simulink model "reduce_emf_load_fixed_v13"  (R2024b)
settings: Solver=FixedStepAuto  StartTime=0.0  StopTime=25  FixedStep=Tsim  RelTol=1e-4  EnableMultiTasking=on
InitFcn:
  | clc;
  | clear;
  | %% Parameters of the motor
  | Tsim = 1e-6;
  | Tpwm=1e-4;
  | Ts = 1e-4;
  | R = 1.8665;
  | Rs=1.8665;
  | Ls=8.96e-3;
  | Ld = 8.96e-3;
  | Lq = 8.96e-3;
  | L1=(Ld +Lq )/2;
  | L2=(Lq -Ld )/2;
  | flux = 0.21;
  | F=0.00008;
  | J=0.003;
  | Np=4;
  | fpwm = 10e3;
  | Vdc=311;
  | wn=100;
  | %% Controller limiter                                                           % Maximum torque (Nm)
  | I_max = 7.5;                                                    % Maximum current (A)
  | V_max = Vdc/sqrt(3);
  | 
  | 
  | %% 转速环电流环带宽
  | wspd=20;
  | wcur=500;
  | 
  | %% LESO
  | w0=10000;
  | beta1=2*w0-R/Ld;
  | beta2=w0*w0;
  | %% IF启动
  | Iq_if=7;
  | we_if_acc=300;
  | we_if_max=180;
  | we_switch=150;
model workspace (MAT data in the model file):
  new = 0
undefined symbols (not defined in the file or in its folder): DiscIntNeverNeededParam
libraries: spsDCVoltageSourceLib x1, spsGroundLib x1, spsPermanentMagnetSynchronousMachineLib x1, spsUniversalBridgeLib x1, spspowerguiLib x1, simulink x1
(part 1 of 2)
settings Model: SimulationMode=accelerator  Creator=Lenovo  LastModifiedBy=azx
settings SolverCC: AlgebraicLoopSolver=TrustRegion
settings DataIOCC: ReturnWorkspaceOutputs=off
settings OptimizationCC: ReuseModelBlockBuffer=off
settings DebuggingCC: UnconnectedInputMsg=warning  UnconnectedOutputMsg=warning  UnconnectedLineMsg=warning
settings ModelReferenceCC: EnableRefExpFcnMdlSchedulingChecks=on
settings RTWCC: GPUComputeCapability=3.5

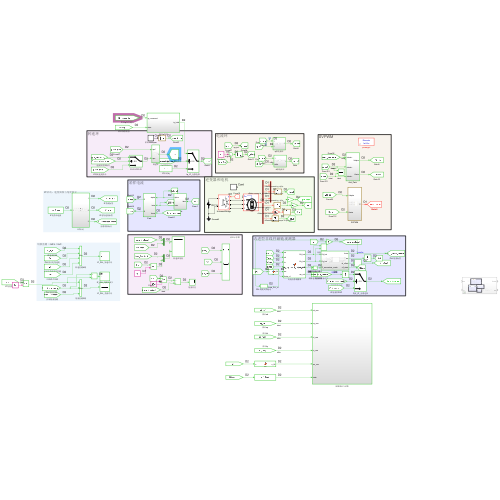
[thumbnail: Simulink's stored preview of the top-level diagram]
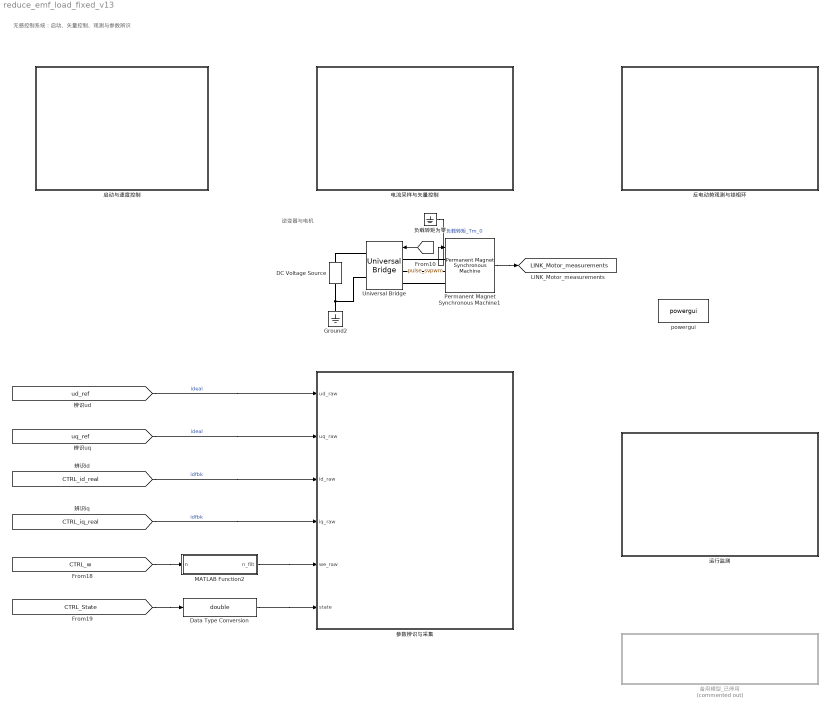
== system reduce_emf_load_fixed_v13 ==
  note: 无感控制系统：启动、矢量控制、观测与参数辨识
  note: 逆变器与电机
  DC Voltage Source : spsDCVoltageSourceLib/DC Voltage Source  Amplitude=Vdc  Measurements=None
  Data Type Conversion : DataTypeConversion  OutDataTypeStr=double  SaturateOnIntegerOverflow=off  RndMeth=Floor
  Ground2 : spsGroundLib/Ground  LConnTagsString=a
  MATLAB Function2 : MATLAB Function  TreatAsAtomicUnit=on
  Permanent Magnet Synchronous Machine1 : spsPermanentMagnetSynchronousMachineLib/Permanent Magnet Synchronous Machine  NbPhases=3  FluxDistribution=Sinusoidal  RotorType=Salient-pole  MechanicalLoad=Torque Tm  PresetModel=No  ShowDetailedParameters=on  MeasurementBus=off  Resistance=R  Inductance=8.5e-3  dqInductances=[Ld,Lq]  La=Ld  MachineConstant=Flux linkage established by magnets (V.s)  Flux=0.21  VoltageCst=152.3591  TorqueCst=1.26  Flat=120  Mechanical=[0.03 2e-2 Np 0]  PolePairs=4  InitialConditions=[0,0, 0,0]  InitialConditions5ph=[0 0 0 0 0 0]  RefAngle=Aligned with phase A axis (original Park)  IterativeDiscreteModel=Trapezoidal non iterative  TsBlock=-1  TsPowergui=0
  Universal Bridge : spsUniversalBridgeLib/Universal Bridge  Arms=3  SnubberResistance=1e5  SnubberCapacitance=inf  Device=IGBT / Diodes  Ron=1e-3  Lon=0  ForwardVoltages="[  0  0  ]"  ForwardVoltage=0  GTOparameters=[ 10e-6 , 20e-6 ]  IGBTparameters=[ 1e-6 , 2e-6 ]  Measurements=None  Measurements_2=None  converterType=Rectifier
  powergui : spspowerguiLib/powergui  Priority=1  SimulationMode=Discrete  SampleTime=Tsim  frequency=60  Iterations=50  frequencyindice=0  Pbase=100e6  ErrMax=1e-4  UnitsV=kV  UnitsW=MW  buscounter=0  FunctionMessages=off  echomessages=off  EnableUseOfTLC=off  CurrentSourceSwitches=off  DisableSnubberDevices=off  DisableRonSwitches=off  DisableVfSwitches=off  DisplayEquations=off  AutomaticDiscreteSolvers=off  SolverType=Tustin/Backward Euler (TBE)  Interpol=off  ExternalGateDelay=off  methode=off  Ts=100  x0status=blocks  SPID=on  SwTol=0  HookPort=off  NonlinearTolerance=1e-4  nMaxIteration=100  ContinueOnMaxIteration=off  RestoreLinks=warning  ResistiveCurrentMeasurement=off  Frange=[0:2:500]  Ylog=off  Xlog=on  ShowGrid=off  save=off  variable=ZData  structure=0  ZoomFFT=off  StartTime=0.0  cycles=1  DisplayStyle=1  fundamental=60  FreqAxis=off  MaxFrequency=1000  frequencyindicesteady=1  RmsSteady=1  display=off
  参数辨识与采集 : Subsystem
  启动与速度控制 : Subsystem  Description=仅整理原计算块与信号标签；虚拟子系统，不增加采样、延迟或执行条件。
  电流采样与矢量控制 : Subsystem  Description=仅整理原计算块与信号标签；虚拟子系统，不增加采样、延迟或执行条件。
  反电动势观测与锁相环 : Subsystem  Description=仅整理原计算块与信号标签；虚拟子系统，不增加采样、延迟或执行条件。
  运行监测 : Subsystem  Description=仅整理原计算块与信号标签；虚拟子系统，不增加采样、延迟或执行条件。
  负载转矩为零 : Ground
  备用模型_已停用 : Subsystem  Commented=on
  tag scope: LINK_Motor_measurements=global
  wires:
  [pulse_svpwm] -> Universal Bridge/1
  Permanent Magnet Synchronous Machine1/1 -> [LINK_Motor_measurements]
  [CTRL_w] -> MATLAB Function2/1(n)
  [CTRL_State] -> Data Type Conversion/1
  [ud_ref] -> 参数辨识与采集/1(ud_raw)  "ideal"
  [uq_ref] -> 参数辨识与采集/2(uq_raw)  "ideal"
  [CTRL_id_real] -> 参数辨识与采集/3(id_raw)  "idfbk"
  [CTRL_iq_real] -> 参数辨识与采集/4(iq_raw)  "idfbk"
  MATLAB Function2/1(n_filt) -> 参数辨识与采集/5(we_raw)
  Data Type Conversion/1 -> 参数辨识与采集/6(state)
  负载转矩为零/1 -> Permanent Magnet Synchronous Machine1/1  "负载转矩_Tm_0"
  connections:
  DC Voltage Source/RConn1 -- Universal Bridge/RConn1
  Permanent Magnet Synchronous Machine1/LConn1 -- Universal Bridge/LConn1
  Permanent Magnet Synchronous Machine1/LConn2 -- Universal Bridge/LConn2
  Permanent Magnet Synchronous Machine1/LConn3 -- Universal Bridge/LConn3
  Universal Bridge/RConn2 -- DC Voltage Source/LConn1 -- Ground2/LConn1

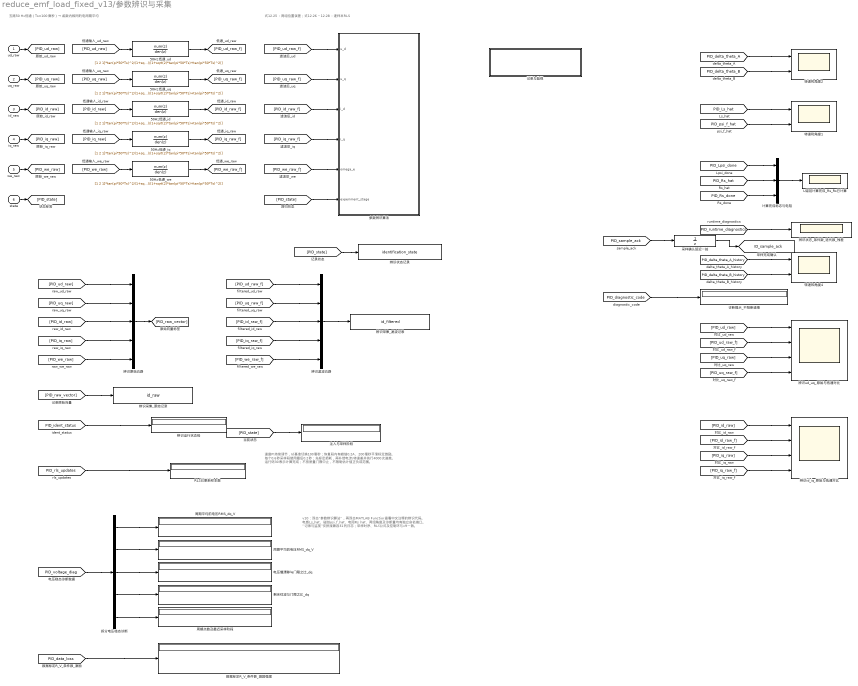
== system reduce_emf_load_fixed_v13/参数辨识与采集 ==
  note: 五路50 Hz低通（Ts=100微秒）→ 函数内相同的电周期平均
  note: 式12.25：两组位置误差；式12.26～12.28：逐样本RLS
  note: 速度PI持续调节，Id基准切换100毫秒；恢复段内有峰值0.2A、200毫秒平滑标定激励。
      | 每个0.6秒采样段使用最后0.2秒；先标定损耗，再补偿电流/转速差并执行4000次递推。
      | 运行码30表示计算完成；不按质量门限中止，不限制估计值正负或范围。
  note: v10：双击“参数辨识算法”，再双击MATLAB Function查看中文注释的辨识代码。
      | 电感Ls_hat、磁链psi_f_hat、电阻Rs_hat、两组角度及诊断量均有独立命名端口。
      | “记录与监视”仅拼接兼容31列日志；采样时序、RLS公式及控制环与v9一致。
  ud_raw : Inport
  uq_raw : Inport  Port=2
  id_raw : Inport  Port=3
  iq_raw : Inport  Port=4
  we_raw : Inport  Port=5
  state : Inport  Port=6
  50Hz低通_id : DiscreteTransferFcn  Description=输入已是Ts=100us；同速率二阶Butterworth低通，不作升采样，不声称恢复上游已混叠信息。  Numerator=[1 2 1]*tan(pi*50*Ts)^2/(1+sqrt(2)*tan(pi*50*Ts)+tan(pi*50*Ts)^2)  Denominator=[1 2*(tan(pi*50*Ts)^2-1)/(1+sqrt(2)*tan(pi*50*Ts)+tan(pi*50*Ts)^2) (1-sqrt(2)*tan(pi*50*Ts)+tan(pi*50*Ts)^2)/(1+sqrt(2)*tan(pi*50*Ts)+tan(pi*50*Ts)^2)]  SampleTime=Ts
  50Hz低通_iq : DiscreteTransferFcn  Description=输入已是Ts=100us；同速率二阶Butterworth低通，不作升采样，不声称恢复上游已混叠信息。  Numerator=[1 2 1]*tan(pi*50*Ts)^2/(1+sqrt(2)*tan(pi*50*Ts)+tan(pi*50*Ts)^2)  Denominator=[1 2*(tan(pi*50*Ts)^2-1)/(1+sqrt(2)*tan(pi*50*Ts)+tan(pi*50*Ts)^2) (1-sqrt(2)*tan(pi*50*Ts)+tan(pi*50*Ts)^2)/(1+sqrt(2)*tan(pi*50*Ts)+tan(pi*50*Ts)^2)]  SampleTime=Ts
  50Hz低通_ud : DiscreteTransferFcn  Description=输入已是Ts=100us；同速率二阶Butterworth低通，不作升采样，不声称恢复上游已混叠信息。  Numerator=[1 2 1]*tan(pi*50*Ts)^2/(1+sqrt(2)*tan(pi*50*Ts)+tan(pi*50*Ts)^2)  Denominator=[1 2*(tan(pi*50*Ts)^2-1)/(1+sqrt(2)*tan(pi*50*Ts)+tan(pi*50*Ts)^2) (1-sqrt(2)*tan(pi*50*Ts)+tan(pi*50*Ts)^2)/(1+sqrt(2)*tan(pi*50*Ts)+tan(pi*50*Ts)^2)]  SampleTime=Ts
  50Hz低通_uq : DiscreteTransferFcn  Description=输入已是Ts=100us；同速率二阶Butterworth低通，不作升采样，不声称恢复上游已混叠信息。  Numerator=[1 2 1]*tan(pi*50*Ts)^2/(1+sqrt(2)*tan(pi*50*Ts)+tan(pi*50*Ts)^2)  Denominator=[1 2*(tan(pi*50*Ts)^2-1)/(1+sqrt(2)*tan(pi*50*Ts)+tan(pi*50*Ts)^2) (1-sqrt(2)*tan(pi*50*Ts)+tan(pi*50*Ts)^2)/(1+sqrt(2)*tan(pi*50*Ts)+tan(pi*50*Ts)^2)]  SampleTime=Ts
  50Hz低通_we : DiscreteTransferFcn  Description=输入已是Ts=100us；同速率二阶Butterworth低通，不作升采样，不声称恢复上游已混叠信息。  Numerator=[1 2 1]*tan(pi*50*Ts)^2/(1+sqrt(2)*tan(pi*50*Ts)+tan(pi*50*Ts)^2)  Denominator=[1 2*(tan(pi*50*Ts)^2-1)/(1+sqrt(2)*tan(pi*50*Ts)+tan(pi*50*Ts)^2) (1-sqrt(2)*tan(pi*50*Ts)+tan(pi*50*Ts)^2)/(1+sqrt(2)*tan(pi*50*Ts)+tan(pi*50*Ts)^2)]  SampleTime=Ts
  L磁链计算完成_Rs_Rs已计算 : Scope
  RLS已更新样本数 : Display
  剩余纹波与门限之比_dq : Display
  周期平均前电压RMS_dq_V : Display
  周期平均后电压RMS_dq_V : Display
  周期点数及最近采样阶段 : Display
  拆分电压稳态诊断 : Demux  Outputs=[2 2 2 2 2]
  注入与采样阶段 : Display
  电压慢漂移与门限之比_dq : Display
  计算完成标志与电阻 : Mux  Inputs=3
  诊断提示_不阻断递推 : Display
  转速和角度1 : Scope  NumInputPorts=2
  转速和角度2 : Scope  NumInputPorts=2
  转速和角度4 : Scope  NumInputPorts=2
  辨识id_iq_原始与低通对比 : Scope
  辨识ud_uq_原始与低通对比 : Scope
  辨识原始五路 : Mux  Inputs=5
  辨识滤波五路 : Mux  Inputs=5
  辨识状态_条件数_迭代数_残差 : Scope
  辨识状态记录 : ToWorkspace  VariableName=identification_state  SaveFormat=Structure With Time  SampleTime=Ts
  辨识运行状态码 : Display
  辨识采集_原始记录 : ToWorkspace  VariableName=id_raw  SaveFormat=Structure With Time  SampleTime=Ts
  辨识采集_滤波记录 : ToWorkspace  VariableName=id_filtered  SaveFormat=Structure With Time  SampleTime=Ts
  采样确认延迟一拍 : UnitDelay  SampleTime=Ts
  数据标定R_V_条件数_激励强度 : Display
  参数辨识算法 : Subsystem
  记录与监视 : Subsystem  Description=将命名信号组合为兼容日志及分组诊断；电感、电阻、磁链直接从各自命名输出读取。
  tag scope: ID_sample_ack=global
  wires:
  [PID_state] -> 辨识状态记录/1
  [PID_delta_theta_A] -> 转速和角度2/1
  [PID_delta_theta_B] -> 转速和角度2/2
  [PID_Ls_hat] -> 转速和角度1/1
  [PID_psi_f_hat] -> 转速和角度1/2
  [PID_Lpsi_done] -> 计算完成标志与电阻/1
  [PID_Rs_hat] -> 计算完成标志与电阻/2
  [PID_Rs_done] -> 计算完成标志与电阻/3
  计算完成标志与电阻/1 -> L磁链计算完成_Rs_Rs已计算/1
  [PID_runtime_diagnostics] -> 辨识状态_条件数_迭代数_残差/1
  [PID_delta_theta_A_history] -> 转速和角度4/1
  [PID_delta_theta_B_history] -> 转速和角度4/2
  [PID_ud_raw] -> 辨识原始五路/1
  [PID_uq_raw] -> 辨识原始五路/2
  [PID_id_raw] -> 辨识原始五路/3
  [PID_iq_raw] -> 辨识原始五路/4
  [PID_we_raw] -> 辨识原始五路/5
  辨识滤波五路/1 -> 辨识采集_滤波记录/1
  [PID_ud_raw_f] -> 辨识滤波五路/1
  [PID_uq_raw_f] -> 辨识滤波五路/2
  [PID_id_raw_f] -> 辨识滤波五路/3
  [PID_iq_raw_f] -> 辨识滤波五路/4
  [PID_we_raw_f] -> 辨识滤波五路/5
  [PID_ud_raw] -> 辨识ud_uq_原始与低通对比/1
  [PID_ud_raw_f] -> 辨识ud_uq_原始与低通对比/2
  [PID_uq_raw] -> 辨识ud_uq_原始与低通对比/3
  [PID_uq_raw_f] -> 辨识ud_uq_原始与低通对比/4
  [PID_id_raw] -> 辨识id_iq_原始与低通对比/1
  [PID_id_raw_f] -> 辨识id_iq_原始与低通对比/2
  [PID_iq_raw] -> 辨识id_iq_原始与低通对比/3
  [PID_iq_raw_f] -> 辨识id_iq_原始与低通对比/4
  辨识原始五路/1 -> [PID_raw_vector]
  [PID_raw_vector] -> 辨识采集_原始记录/1
  采样确认延迟一拍/1 -> [ID_sample_ack]
  [PID_state] -> 注入与采样阶段/1
  ud_raw/1 -> [PID_ud_raw]
  [PID_ud_raw] -> 50Hz低通_ud/1
  50Hz低通_ud/1 -> [PID_ud_raw_f]
  uq_raw/1 -> [PID_uq_raw]
  [PID_uq_raw] -> 50Hz低通_uq/1
  50Hz低通_uq/1 -> [PID_uq_raw_f]
  id_raw/1 -> [PID_id_raw]
  [PID_id_raw] -> 50Hz低通_id/1
  50Hz低通_id/1 -> [PID_id_raw_f]
  iq_raw/1 -> [PID_iq_raw]
  [PID_iq_raw] -> 50Hz低通_iq/1
  50Hz低通_iq/1 -> [PID_iq_raw_f]
  we_raw/1 -> [PID_we_raw]
  [PID_we_raw] -> 50Hz低通_we/1
  50Hz低通_we/1 -> [PID_we_raw_f]
  state/1 -> [PID_state]
  [PID_voltage_diag] -> 拆分电压稳态诊断/1
  拆分电压稳态诊断/1 -> 周期平均前电压RMS_dq_V/1
  拆分电压稳态诊断/2 -> 周期平均后电压RMS_dq_V/1
  拆分电压稳态诊断/3 -> 电压慢漂移与门限之比_dq/1
  拆分电压稳态诊断/4 -> 剩余纹波与门限之比_dq/1
  拆分电压稳态诊断/5 -> 周期点数及最近采样阶段/1
  [PID_data_loss] -> 数据标定R_V_条件数_激励强度/1
  [PID_ud_raw_f] -> 参数辨识算法/1(u_d)
  [PID_uq_raw_f] -> 参数辨识算法/2(u_q)
  [PID_id_raw_f] -> 参数辨识算法/3(i_d)
  [PID_iq_raw_f] -> 参数辨识算法/4(i_q)
  [PID_we_raw_f] -> 参数辨识算法/5(omega_e)
  [PID_state] -> 参数辨识算法/6(experiment_stage)
  [PID_sample_ack] -> 采样确认延迟一拍/1
  [PID_diagnostic_code] -> 诊断提示_不阻断递推/1
  [PID_ident_status] -> 辨识运行状态码/1
  [PID_rls_updates] -> RLS已更新样本数/1

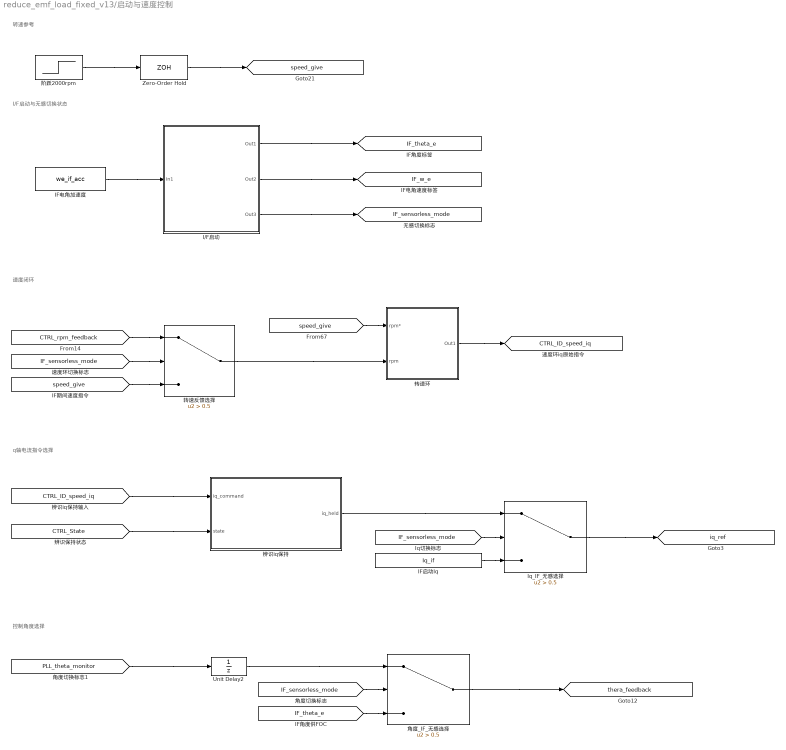
== system reduce_emf_load_fixed_v13/启动与速度控制 ==
  note: 转速参考
  note: I/F启动与无感切换状态
  note: 速度闭环
  note: q轴电流指令选择
  note: 控制角度选择
  阶跃2000rpm : Step  Time=2  Before=500  After=500  SampleTime=0
  Zero-Order Hold : ZeroOrderHold  SampleTime=1e-4
  IF电角加速度 : Constant  Value=we_if_acc  SampleTime=Ts
  I/F启动 : Subsystem
  转速环 : Subsystem
  转速反馈选择 : Switch  Criteria=u2 > Threshold  Threshold=0.5
  辨识iq保持 : Subsystem
  Iq_IF_无感选择 : Switch  Criteria=u2 > Threshold  Threshold=0.5
  IF启动Iq : Constant  Value=Iq_if  SampleTime=Ts
  Unit Delay2 : UnitDelay  SampleTime=-1  HasFrameUpgradeWarning=on
  角度_IF_无感选择 : Switch  Criteria=u2 > Threshold  Threshold=0.5
  tag scope: CTRL_ID_speed_iq=global, IF_sensorless_mode=global, IF_theta_e=global, IF_w_e=global, iq_ref=global, speed_give=global, thera_feedback=global
  wires:
  Zero-Order Hold/1 -> [speed_give]
  角度_IF_无感选择/1 -> [thera_feedback]
  Iq_IF_无感选择/1 -> [iq_ref]
  I/F启动/1(Out1) -> [IF_theta_e]
  I/F启动/2(Out2) -> [IF_w_e]
  I/F启动/3(Out3) -> [IF_sensorless_mode]
  转速环/1(Out1) -> [CTRL_ID_speed_iq]
  阶跃2000rpm/1 -> Zero-Order Hold/1
  [speed_give] -> 转速环/1(rpm*)
  [IF_sensorless_mode] -> Iq_IF_无感选择/2
  IF启动Iq/1 -> Iq_IF_无感选择/3
  [CTRL_rpm_feedback] -> 转速反馈选择/1
  [IF_sensorless_mode] -> 转速反馈选择/2
  [speed_give] -> 转速反馈选择/3
  转速反馈选择/1 -> 转速环/2(rpm)
  [IF_sensorless_mode] -> 角度_IF_无感选择/2
  [IF_theta_e] -> 角度_IF_无感选择/3
  [PLL_theta_monitor] -> Unit Delay2/1
  IF电角加速度/1 -> I/F启动/1(In1)
  Unit Delay2/1 -> 角度_IF_无感选择/1
  [CTRL_State] -> 辨识iq保持/2(state)
  辨识iq保持/1(iq_held) -> Iq_IF_无感选择/1
  [CTRL_ID_speed_iq] -> 辨识iq保持/1(iq_command)

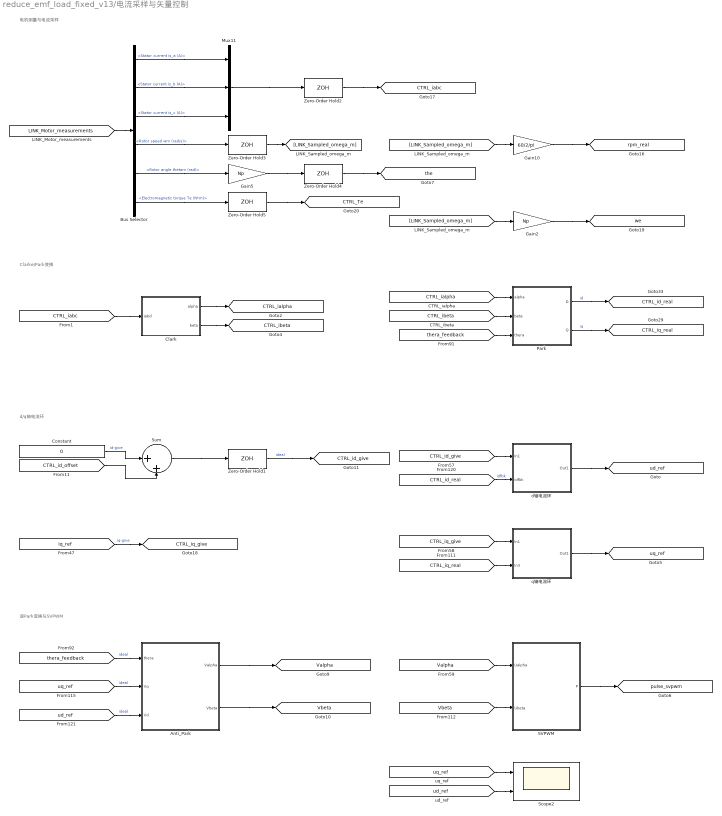
== system reduce_emf_load_fixed_v13/电流采样与矢量控制 ==
  note: 电机测量与电流采样
  note: Clarke/Park变换
  note: d/q轴电流环
  note: 逆Park变换与SVPWM
  Bus Selector : BusSelector  OutputSignals=Stator current is_a (A),Stator current is_b (A),Stator current is_c (A),Rotor speed wm (rad/s),Rotor angle thetam (rad),Electromagnetic torque Te (N*m)
  Mux11 : Mux  Inputs=3
  Zero-Order Hold{1..5} (5 alike) : ZeroOrderHold  SampleTime=1e-4
  Gain10 : Gain  Gain=60/2/pi
  Gain2 : Gain  Gain=Np
  Gain5 : Gain  Gain=Np
  Clark : Subsystem
  Park : Subsystem
  Constant : Constant  Value=0
  Sum : Sum  Inputs=|++
  d轴电流环 : Subsystem
  q轴电流环 : Subsystem
  Anti_Park : Subsystem
  SVPWM : Subsystem
  Scope2 : Scope  NumInputPorts=2
  tag scope: CTRL_Te=global, CTRL_iabc=global, CTRL_ialpha=global, CTRL_ibeta=global, CTRL_id_give=global, CTRL_id_real=global, CTRL_iq_give=global, CTRL_iq_real=global, Valpha=global, Vbeta=global, pulse_svpwm=global, rpm_real=global, the=global, ud_ref=global, uq_ref=global, we=global
  wires:
  Clark/2(beta) -> [CTRL_ibeta]
  Clark/1(alpha) -> [CTRL_ialpha]
  Park/1(D) -> [CTRL_id_real]  "id"
  Park/2(Q) -> [CTRL_iq_real]  "iq"
  Zero-Order Hold1/1 -> [CTRL_id_give]  "ideal"
  Zero-Order Hold5/1 -> [CTRL_Te]
  Gain2/1 -> [we]
  Zero-Order Hold2/1 -> [CTRL_iabc]
  Gain10/1 -> [rpm_real]
  Zero-Order Hold4/1 -> [the]
  Anti_Park/1(Valpha) -> [Valpha]
  Anti_Park/2(Vbeta) -> [Vbeta]
  q轴电流环/1(Out1) -> [uq_ref]
  d轴电流环/1(Out1) -> [ud_ref]
  SVPWM/1(P) -> [pulse_svpwm]
  [iq_ref] -> [CTRL_iq_give]  "iq-give"
  [CTRL_ibeta] -> Park/2(beta)
  [CTRL_ialpha] -> Park/1(alpha)
  [thera_feedback] -> Park/3(thera)
  [thera_feedback] -> Anti_Park/1(thera)  "ideal"
  [ud_ref] -> Scope2/2
  [ud_ref] -> Anti_Park/3(Vd)  "ideal"
  [uq_ref] -> Scope2/1
  [uq_ref] -> Anti_Park/2(Vq)  "ideal"
  [CTRL_iabc] -> Clark/1(iabd)
  Bus Selector/1 -> Mux11/1  "<Stator current is_a (A)>"
  Bus Selector/3 -> Mux11/3  "<Stator current is_c (A)>"
  Zero-Order Hold3/1 -> [LINK_Sampled_omega_m]
  [LINK_Sampled_omega_m] -> Gain2/1
  [LINK_Sampled_omega_m] -> Gain10/1
  Mux11/1 -> Zero-Order Hold2/1
  Bus Selector/2 -> Mux11/2  "<Stator current is_b (A)>"
  Bus Selector/5 -> Gain5/1  "<Rotor angle thetam (rad)>"
  Bus Selector/4 -> Zero-Order Hold3/1  "<Rotor speed wm (rad/s)>"
  Bus Selector/6 -> Zero-Order Hold5/1  "<Electromagnetic torque Te (N*m)>"
  [LINK_Motor_measurements] -> Bus Selector/1
  Gain5/1 -> Zero-Order Hold4/1
  [CTRL_iq_give] -> q轴电流环/1(In1)
  [CTRL_iq_real] -> q轴电流环/2(In3)
  [CTRL_id_give] -> d轴电流环/1(In1)
  [CTRL_id_real] -> d轴电流环/2(idfbk)  "idfbk"
  [Valpha] -> SVPWM/1(Ualpha)
  [Vbeta] -> SVPWM/2(Ubeta)
  Sum/1 -> Zero-Order Hold1/1
  Constant/1 -> Sum/1  "id-give"
  [CTRL_id_offset] -> Sum/2

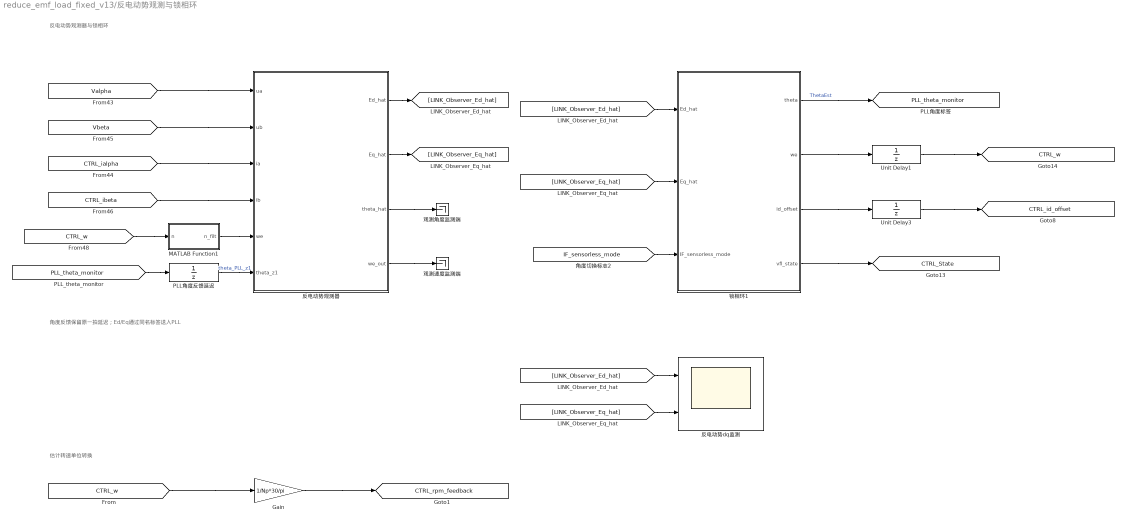
== system reduce_emf_load_fixed_v13/反电动势观测与锁相环 ==
  note: 反电动势观测器与锁相环
  note: 角度反馈保留原一拍延迟；Ed/Eq通过同名标签送入PLL
  note: 估计转速单位转换
  MATLAB Function1 : MATLAB Function  Description=旁路100Hz低通，使用原有一拍延迟PLL速度，与角度反馈推进严格同拍。  TreatAsAtomicUnit=on
  PLL角度反馈延迟 : UnitDelay  SampleTime=1e-4
  反电动势观测器 : MATLAB Function  Description=按文档式12.5-12.7、图12.2实现dq降阶反电动势观测器，Ed/Eq直接送PLL。  TreatAsAtomicUnit=on
  锁相环1 : Subsystem  Description=v9：速度PI不冻结；采样段0.6秒，Id恢复段1秒含0.2A平滑标定激励，正式采样前恢复650毫秒。
  Unit Delay1 : UnitDelay  SampleTime=-1  HasFrameUpgradeWarning=on
  Unit Delay3 : UnitDelay  SampleTime=-1  HasFrameUpgradeWarning=on
  观测角度监测端 : Terminator
  观测速度监测端 : Terminator
  反电动势dq监测 : Scope  NumInputPorts=2
  Gain : Gain  Gain=1/Np*30/pi
  tag scope: CTRL_State=global, CTRL_id_offset=global, CTRL_rpm_feedback=global, CTRL_w=global, PLL_theta_monitor=global
  wires:
  Gain/1 -> [CTRL_rpm_feedback]
  Unit Delay1/1 -> [CTRL_w]
  锁相环1/1(theta) -> [PLL_theta_monitor]  "ThetaEst"
  Unit Delay3/1 -> [CTRL_id_offset]
  锁相环1/4(vfl_state) -> [CTRL_State]
  [Valpha] -> 反电动势观测器/1(ua)
  反电动势观测器/2(Eq_hat) -> [LINK_Observer_Eq_hat]
  [LINK_Observer_Eq_hat] -> 锁相环1/2(Eq_hat)
  [LINK_Observer_Eq_hat] -> 反电动势dq监测/2
  [Vbeta] -> 反电动势观测器/2(ub)
  [CTRL_ialpha] -> 反电动势观测器/3(ia)
  [CTRL_ibeta] -> 反电动势观测器/4(ib)
  反电动势观测器/1(Ed_hat) -> [LINK_Observer_Ed_hat]
  [LINK_Observer_Ed_hat] -> 锁相环1/1(Ed_hat)
  [LINK_Observer_Ed_hat] -> 反电动势dq监测/1
  锁相环1/2(we) -> Unit Delay1/1
  [CTRL_w] -> MATLAB Function1/1(n)
  [CTRL_w] -> Gain/1
  [PLL_theta_monitor] -> PLL角度反馈延迟/1
  [IF_sensorless_mode] -> 锁相环1/3(IF_sensorless_mode)
  锁相环1/3(id_offset) -> Unit Delay3/1
  MATLAB Function1/1(n_filt) -> 反电动势观测器/5("we ")
  PLL角度反馈延迟/1 -> 反电动势观测器/6(theta_z1)  "theta_PLL_z1"
  反电动势观测器/3(theta_hat) -> 观测角度监测端/1
  反电动势观测器/4(we_out) -> 观测速度监测端/1

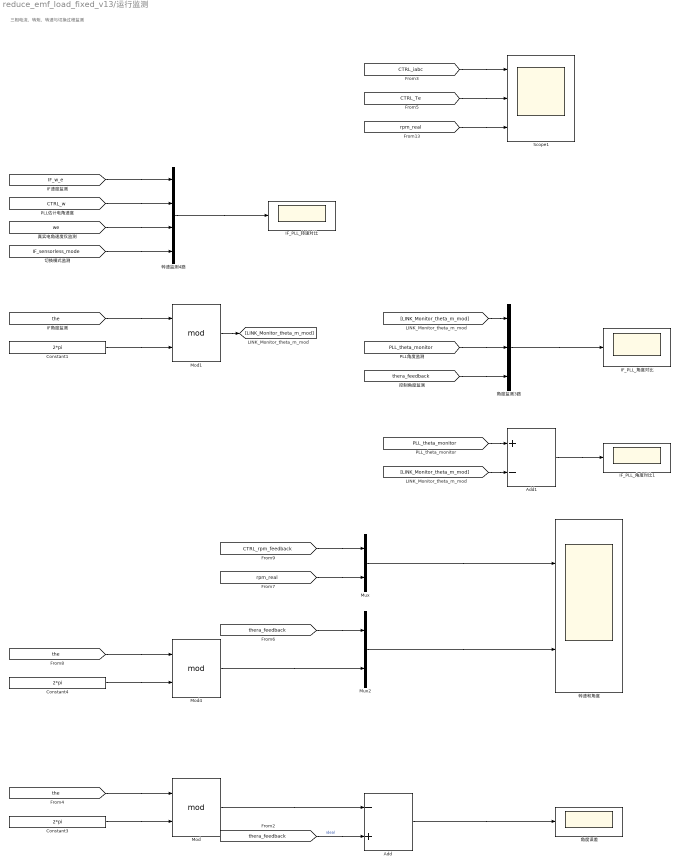
== system reduce_emf_load_fixed_v13/运行监测 ==
  note: 三相电流、转矩、转速与切换过程监测
  Scope1 : Scope  NumInputPorts=3
  转速监测4路 : Mux
  IF_PLL_转速对比 : Scope
  Constant1 : Constant  Value=2*pi
  Mod1 : Math  Operator=mod
  角度监测3路 : Mux  Inputs=3
  IF_PLL_角度对比 : Scope
  Add1 : Sum  Inputs=+-
  IF_PLL_角度对比1 : Scope
  Mux : Mux  Inputs=2
  Mux2 : Mux  Inputs=2
  转速和角度 : Scope  NumInputPorts=2
  Constant4 : Constant  Value=2*pi
  Mod4 : Math  Operator=mod
  Constant3 : Constant  Value=2*pi
  Mod : Math  Operator=mod
  Add : Sum  Inputs=-+
  角度误差 : Scope
  wires:
  [CTRL_rpm_feedback] -> Mux/1
  [rpm_real] -> Mux/2
  [thera_feedback] -> Mux2/1
  Mux2/1 -> 转速和角度/2
  Mux/1 -> 转速和角度/1
  [the] -> Mod/1
  Constant3/1 -> Mod/2
  Mod/1 -> Add/1
  Add/1 -> 角度误差/1
  [thera_feedback] -> Add/2  "ideal"
  [the] -> Mod4/1
  Constant4/1 -> Mod4/2
  Mod4/1 -> Mux2/2
  [rpm_real] -> Scope1/3
  [CTRL_Te] -> Scope1/2
  [CTRL_iabc] -> Scope1/1
  [IF_w_e] -> 转速监测4路/1
  [CTRL_w] -> 转速监测4路/2
  [we] -> 转速监测4路/3
  [IF_sensorless_mode] -> 转速监测4路/4
  转速监测4路/1 -> IF_PLL_转速对比/1
  [PLL_theta_monitor] -> Add1/1
  [PLL_theta_monitor] -> 角度监测3路/2
  [thera_feedback] -> 角度监测3路/3
  角度监测3路/1 -> IF_PLL_角度对比/1
  Add1/1 -> IF_PLL_角度对比1/1
  [the] -> Mod1/1
  Constant1/1 -> Mod1/2
  Mod1/1 -> [LINK_Monitor_theta_m_mod]
  [LINK_Monitor_theta_m_mod] -> Add1/2
  [LINK_Monitor_theta_m_mod] -> 角度监测3路/1

== system reduce_emf_load_fixed_v13/备用模型_已停用 ==
  Subsystem : Subsystem  Commented=on
  Step1 : Step  Time=0.5  Before=8.5  After=8.5  SampleTime=0
  备用输入1 : Ground
  备用输入2 : Ground
  备用输出1 : Terminator
  备用输出2 : Terminator
  未启用的备用负载 : Terminator
  wires:
  备用输入1/1 -> Subsystem/1(ea)
  备用输入2/1 -> Subsystem/2(eb)
  Subsystem/1(theta) -> 备用输出1/1
  Subsystem/2(we) -> 备用输出2/1
  Step1/1 -> 未启用的备用负载/1

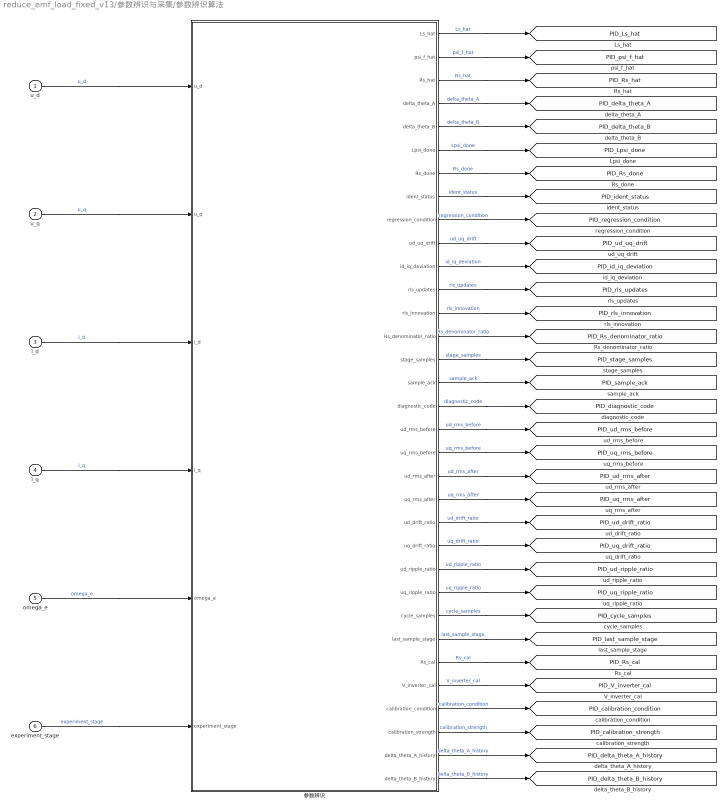
== system reduce_emf_load_fixed_v13/参数辨识与采集/参数辨识算法 ==
  参数辨识 : MATLAB Function  Description=v10：独立命名输出，中文注释；仅重构代码风格及接口，数值算法与v9一致。  TreatAsAtomicUnit=on
  u_d : Inport  Port=1
  u_q : Inport  Port=2
  i_d : Inport  Port=3
  i_q : Inport  Port=4
  omega_e : Inport  Port=5
  experiment_stage : Inport  Port=6
  tag scope: PID_Lpsi_done=global, PID_Ls_hat=global, PID_Rs_cal=global, PID_Rs_denominator_ratio=global, PID_Rs_done=global, PID_Rs_hat=global, PID_V_inverter_cal=global, PID_calibration_condition=global, PID_calibration_strength=global, PID_cycle_samples=global, PID_delta_theta_A=global, PID_delta_theta_A_history=global, PID_delta_theta_B=global, PID_delta_theta_B_history=global, PID_diagnostic_code=global, PID_id_iq_deviation=global, PID_ident_status=global, PID_last_sample_stage=global, PID_psi_f_hat=global, PID_regression_condition=global, PID_rls_innovation=global, PID_rls_updates=global, PID_sample_ack=global, PID_stage_samples=global, PID_ud_drift_ratio=global, PID_ud_ripple_ratio=global, PID_ud_rms_after=global, PID_ud_rms_before=global, PID_ud_uq_drift=global, PID_uq_drift_ratio=global, PID_uq_ripple_ratio=global, PID_uq_rms_after=global, PID_uq_rms_before=global
  wires:
  u_d/1 -> 参数辨识/1(u_d)  "u_d"
  u_q/1 -> 参数辨识/2(u_q)  "u_q"
  i_d/1 -> 参数辨识/3(i_d)  "i_d"
  i_q/1 -> 参数辨识/4(i_q)  "i_q"
  omega_e/1 -> 参数辨识/5(omega_e)  "omega_e"
  experiment_stage/1 -> 参数辨识/6(experiment_stage)  "experiment_stage"
  参数辨识/1(Ls_hat) -> [PID_Ls_hat]  "Ls_hat"
  参数辨识/2(psi_f_hat) -> [PID_psi_f_hat]  "psi_f_hat"
  参数辨识/3(Rs_hat) -> [PID_Rs_hat]  "Rs_hat"
  参数辨识/4(delta_theta_A) -> [PID_delta_theta_A]  "delta_theta_A"
  参数辨识/5(delta_theta_B) -> [PID_delta_theta_B]  "delta_theta_B"
  参数辨识/6(Lpsi_done) -> [PID_Lpsi_done]  "Lpsi_done"
  参数辨识/7(Rs_done) -> [PID_Rs_done]  "Rs_done"
  参数辨识/8(ident_status) -> [PID_ident_status]  "ident_status"
  参数辨识/9(regression_condition) -> [PID_regression_condition]  "regression_condition"
  参数辨识/10(ud_uq_drift) -> [PID_ud_uq_drift]  "ud_uq_drift"
  参数辨识/11(id_iq_deviation) -> [PID_id_iq_deviation]  "id_iq_deviation"
  参数辨识/12(rls_updates) -> [PID_rls_updates]  "rls_updates"
  参数辨识/13(rls_innovation) -> [PID_rls_innovation]  "rls_innovation"
  参数辨识/14(Rs_denominator_ratio) -> [PID_Rs_denominator_ratio]  "Rs_denominator_ratio"
  参数辨识/15(stage_samples) -> [PID_stage_samples]  "stage_samples"
  参数辨识/16(sample_ack) -> [PID_sample_ack]  "sample_ack"
  参数辨识/17(diagnostic_code) -> [PID_diagnostic_code]  "diagnostic_code"
  参数辨识/18(ud_rms_before) -> [PID_ud_rms_before]  "ud_rms_before"
  参数辨识/19(uq_rms_before) -> [PID_uq_rms_before]  "uq_rms_before"
  参数辨识/20(ud_rms_after) -> [PID_ud_rms_after]  "ud_rms_after"
  参数辨识/21(uq_rms_after) -> [PID_uq_rms_after]  "uq_rms_after"
  参数辨识/22(ud_drift_ratio) -> [PID_ud_drift_ratio]  "ud_drift_ratio"
  参数辨识/23(uq_drift_ratio) -> [PID_uq_drift_ratio]  "uq_drift_ratio"
  参数辨识/24(ud_ripple_ratio) -> [PID_ud_ripple_ratio]  "ud_ripple_ratio"
  参数辨识/25(uq_ripple_ratio) -> [PID_uq_ripple_ratio]  "uq_ripple_ratio"
  参数辨识/26(cycle_samples) -> [PID_cycle_samples]  "cycle_samples"
  参数辨识/27(last_sample_stage) -> [PID_last_sample_stage]  "last_sample_stage"
  参数辨识/28(Rs_cal) -> [PID_Rs_cal]  "Rs_cal"
  参数辨识/29(V_inverter_cal) -> [PID_V_inverter_cal]  "V_inverter_cal"
  参数辨识/30(calibration_condition) -> [PID_calibration_condition]  "calibration_condition"
  参数辨识/31(calibration_strength) -> [PID_calibration_strength]  "calibration_strength"
  参数辨识/32(delta_theta_A_history) -> [PID_delta_theta_A_history]  "delta_theta_A_history"
  参数辨识/33(delta_theta_B_history) -> [PID_delta_theta_B_history]  "delta_theta_B_history"

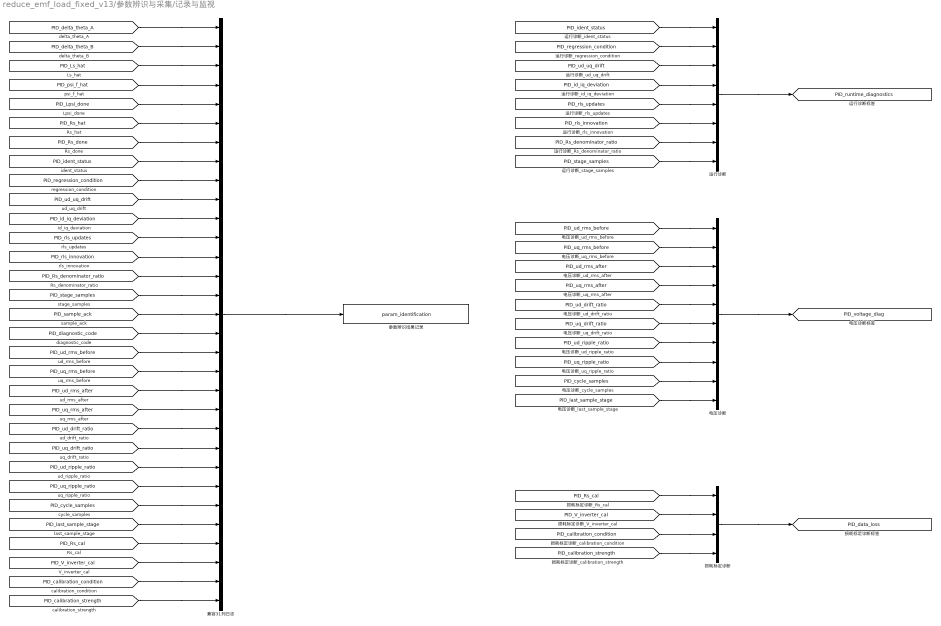
== system reduce_emf_load_fixed_v13/参数辨识与采集/记录与监视 ==
  兼容31列日志 : Mux  Inputs=31
  运行诊断 : Mux  Inputs=8
  电压诊断 : Mux  Inputs=10
  损耗标定诊断 : Mux  Inputs=4
  参数辨识结果记录 : ToWorkspace  VariableName=param_identification  SaveFormat=Structure With Time  SampleTime=Ts
  tag scope: PID_data_loss=global, PID_runtime_diagnostics=global, PID_voltage_diag=global
  wires:
  [PID_delta_theta_A] -> 兼容31列日志/1
  [PID_delta_theta_B] -> 兼容31列日志/2
  [PID_Ls_hat] -> 兼容31列日志/3
  [PID_psi_f_hat] -> 兼容31列日志/4
  [PID_Lpsi_done] -> 兼容31列日志/5
  [PID_Rs_hat] -> 兼容31列日志/6
  [PID_Rs_done] -> 兼容31列日志/7
  [PID_ident_status] -> 兼容31列日志/8
  [PID_regression_condition] -> 兼容31列日志/9
  [PID_ud_uq_drift] -> 兼容31列日志/10
  [PID_id_iq_deviation] -> 兼容31列日志/11
  [PID_rls_updates] -> 兼容31列日志/12
  [PID_rls_innovation] -> 兼容31列日志/13
  [PID_Rs_denominator_ratio] -> 兼容31列日志/14
  [PID_stage_samples] -> 兼容31列日志/15
  [PID_sample_ack] -> 兼容31列日志/16
  [PID_diagnostic_code] -> 兼容31列日志/17
  [PID_ud_rms_before] -> 兼容31列日志/18
  [PID_uq_rms_before] -> 兼容31列日志/19
  [PID_ud_rms_after] -> 兼容31列日志/20
  [PID_uq_rms_after] -> 兼容31列日志/21
  [PID_ud_drift_ratio] -> 兼容31列日志/22
  [PID_uq_drift_ratio] -> 兼容31列日志/23
  [PID_ud_ripple_ratio] -> 兼容31列日志/24
  [PID_uq_ripple_ratio] -> 兼容31列日志/25
  [PID_cycle_samples] -> 兼容31列日志/26
  [PID_last_sample_stage] -> 兼容31列日志/27
  [PID_Rs_cal] -> 兼容31列日志/28
  [PID_V_inverter_cal] -> 兼容31列日志/29
  [PID_calibration_condition] -> 兼容31列日志/30
  [PID_calibration_strength] -> 兼容31列日志/31
  兼容31列日志/1 -> 参数辨识结果记录/1
  [PID_ident_status] -> 运行诊断/1
  [PID_regression_condition] -> 运行诊断/2
  [PID_ud_uq_drift] -> 运行诊断/3
  [PID_id_iq_deviation] -> 运行诊断/4
  [PID_rls_updates] -> 运行诊断/5
  [PID_rls_innovation] -> 运行诊断/6
  [PID_Rs_denominator_ratio] -> 运行诊断/7
  [PID_stage_samples] -> 运行诊断/8
  运行诊断/1 -> [PID_runtime_diagnostics]
  [PID_ud_rms_before] -> 电压诊断/1
  [PID_uq_rms_before] -> 电压诊断/2
  [PID_ud_rms_after] -> 电压诊断/3
  [PID_uq_rms_after] -> 电压诊断/4
  [PID_ud_drift_ratio] -> 电压诊断/5
  [PID_uq_drift_ratio] -> 电压诊断/6
  [PID_ud_ripple_ratio] -> 电压诊断/7
  [PID_uq_ripple_ratio] -> 电压诊断/8
  [PID_cycle_samples] -> 电压诊断/9
  [PID_last_sample_stage] -> 电压诊断/10
  电压诊断/1 -> [PID_voltage_diag]
  [PID_Rs_cal] -> 损耗标定诊断/1
  [PID_V_inverter_cal] -> 损耗标定诊断/2
  [PID_calibration_condition] -> 损耗标定诊断/3
  [PID_calibration_strength] -> 损耗标定诊断/4
  损耗标定诊断/1 -> [PID_data_loss]

== system reduce_emf_load_fixed_v13/启动与速度控制/I//F启动 ==
  In1 : Inport
  2π : Constant  Value=2*pi  SampleTime=Ts
  Data Type Conversion : DataTypeConversion  OutDataTypeStr=double  SaturateOnIntegerOverflow=off  RndMeth=Floor
  IF角度取模 : Math  Operator=mod
  IF角度积分 : DiscreteIntegrator  SampleTime=Ts  ICPrevOutput=DiscIntNeverNeededParam  ICPrevScaledInput=DiscIntNeverNeededParam
  IF转速达到阈值 : RelationalOperator
  IF速度上限 : Saturate  UpperLimit=we_if_max  LowerLimit=0
  IF速度积分 : DiscreteIntegrator  SampleTime=Ts  ICPrevOutput=DiscIntNeverNeededParam  ICPrevScaledInput=DiscIntNeverNeededParam
  切换电角速度 : Constant  Value=we_switch  SampleTime=Ts
  Out1 : Outport
  Out2 : Outport  Port=2
  Out3 : Outport  Port=3
  wires:
  切换电角速度/1 -> IF转速达到阈值/2
  IF速度积分/1 -> IF速度上限/1
  2π/1 -> IF角度取模/2
  IF速度上限/1 -> Out2/1, IF转速达到阈值/1, IF角度积分/1
  IF角度积分/1 -> IF角度取模/1
  IF转速达到阈值/1 -> Data Type Conversion/1
  In1/1 -> IF速度积分/1
  Data Type Conversion/1 -> Out3/1
  IF角度取模/1 -> Out1/1

== system reduce_emf_load_fixed_v13/启动与速度控制/转速环 ==
  rpm* : Inport
  rpm : Inport  Port=2
  30speed : Subsystem  DialogController=POWERSYS.PowerSysDialog  mask(Discrete PI Controller){Kp=0.5, Ki=5, Par_Limits=[I_max -I_max], Init=0, Ts=Ts}
      mask prompts: Kp "Proportional gain (Kp):"; Ki "Integral gain (Ki):"; Par_Limits "Output limits: [ Upper   Lower ]"; Init "Output initial value:"; Ts "Sample time:"
      mask help: This block implements a discrete PI controller.
      mask init:
      | UpperLimit=Par_Limits(1);
      | LowerLimit=Par_Limits(2);
      | power_initmask();
      mask Help: This block is part of a subset of blocks in the Extras library that does not have documentation associated with it, other than the block mask description.
      mask Display: disp('PI');
  Gain : Gain  Gain=2*pi/60
  Sum : Sum  Inputs=|+-
  辨识期间暂停速度PI误差 : Switch  Criteria=u2 > Threshold  Threshold=0.5
  辨识期间零速度误差 : Constant  Value=0  SampleTime=Ts
  Out1 : Outport
  wires:
  Sum/1 -> Gain/1
  rpm*/1 -> Sum/1
  rpm/1 -> Sum/2
  Gain/1 -> 辨识期间暂停速度PI误差/3
  30speed/1(Out) -> Out1/1
  [ID_acquisition_hold] -> 辨识期间暂停速度PI误差/2
  辨识期间零速度误差/1 -> 辨识期间暂停速度PI误差/1
  辨识期间暂停速度PI误差/1 -> 30speed/1(Error)

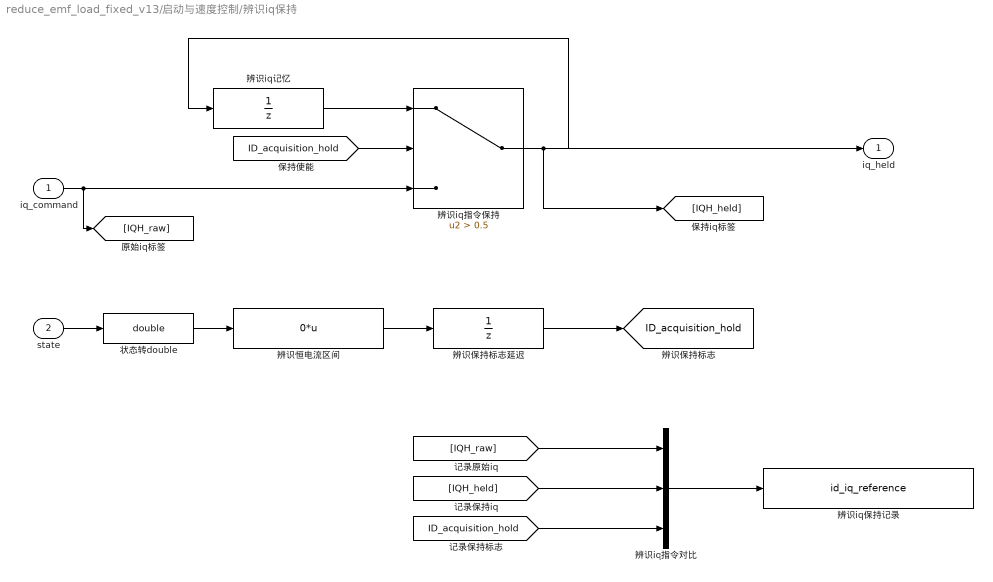
== system reduce_emf_load_fixed_v13/启动与速度控制/辨识iq保持 ==
  iq_command : Inport
  state : Inport  Port=2
  状态转double : DataTypeConversion  OutDataTypeStr=double
  辨识iq保持记录 : ToWorkspace  VariableName=id_iq_reference  SaveFormat=Structure With Time  SampleTime=Ts
  辨识iq指令保持 : Switch  Criteria=u2 > Threshold  Threshold=0.5
  辨识iq指令对比 : Mux  Inputs=3
  辨识iq记忆 : UnitDelay  SampleTime=Ts
  辨识保持标志延迟 : UnitDelay  SampleTime=Ts
  辨识恒电流区间 : Fcn  Expr=0*u  Description=辨识保持使能固定为0：iq直通速度PI输出，速度PI误差不再置零。
  iq_held : Outport
  tag scope: ID_acquisition_hold=global
  wires:
  state/1 -> 状态转double/1
  状态转double/1 -> 辨识恒电流区间/1
  iq_command/1 -> 辨识iq指令保持/3, [IQH_raw]
  辨识恒电流区间/1 -> 辨识保持标志延迟/1
  辨识保持标志延迟/1 -> [ID_acquisition_hold]
  [ID_acquisition_hold] -> 辨识iq指令保持/2
  辨识iq记忆/1 -> 辨识iq指令保持/1
  辨识iq指令保持/1 -> 辨识iq记忆/1, iq_held/1, [IQH_held]
  [IQH_raw] -> 辨识iq指令对比/1
  [IQH_held] -> 辨识iq指令对比/2
  [ID_acquisition_hold] -> 辨识iq指令对比/3
  辨识iq指令对比/1 -> 辨识iq保持记录/1

== system reduce_emf_load_fixed_v13/电流采样与矢量控制/Clark ==
  iabd : Inport
  Fcn : Fcn  Expr=(u(1)-0.5*(u(2)+u(3)))*2/3
  Fcn1 : Fcn  Expr=sqrt(3)/2*(u(2)-u(3))*2/3
  alpha : Outport
  beta : Outport  Port=2
  tag scope: Ialpha_real=global, Ibeta_real=global
  wires:
  iabd/1 -> Fcn1/1, Fcn/1
  Fcn/1 -> [Ialpha_real], alpha/1
  Fcn1/1 -> [Ibeta_real], beta/1

== system reduce_emf_load_fixed_v13/电流采样与矢量控制/Park ==
  alpha : Inport
  beta : Inport  Port=2
  thera : Inport  Port=3
  Fcn : Fcn  Expr=u(1)*cos(u(3))+u(2)*sin(u(3))
  Fcn1 : Fcn  Expr=-u(1)*sin(u(3))+u(2)*cos(u(3))
  Mux1 : Mux  Inputs=3
  D : Outport
  Q : Outport  Port=2
  wires:
  beta/1 -> Mux1/2
  Mux1/1 -> Fcn1/1, Fcn/1
  thera/1 -> Mux1/3
  Fcn/1 -> D/1
  Fcn1/1 -> Q/1
  alpha/1 -> Mux1/1

== system reduce_emf_load_fixed_v13/电流采样与矢量控制/d轴电流环 ==
  In1 : Inport
  idfbk : Inport  Port=2
  30id : Subsystem  DialogController=POWERSYS.PowerSysDialog  mask(Discrete PI Controller){Kp=2*pi*wcur*Ld, Ki=2*pi*wcur*R, Par_Limits=[V_max -V_max], Init=0, Ts=Ts}
      mask prompts: Kp "Proportional gain (Kp):"; Ki "Integral gain (Ki):"; Par_Limits "Output limits: [ Upper   Lower ]"; Init "Output initial value:"; Ts "Sample time:"
      mask help: This block implements a discrete PI controller.
      mask init:
      | UpperLimit=Par_Limits(1);
      | LowerLimit=Par_Limits(2);
      | power_initmask();
      mask Help: This block is part of a subset of blocks in the Extras library that does not have documentation associated with it, other than the block mask description.
      mask Display: disp('PI');
  Sum1 : Sum  Inputs=|+-
  Sum7 : Sum  Inputs=|+-
  Out1 : Outport
  wires:
  30id/1(Out) -> Sum7/1  "ideal"
  Sum1/1 -> 30id/1(Error)
  Sum7/1 -> Out1/1
  idfbk/1 -> Sum1/2
  In1/1 -> Sum1/1

== system reduce_emf_load_fixed_v13/电流采样与矢量控制/q轴电流环 ==
  In1 : Inport
  In3 : Inport  Port=2
  30iq : Subsystem  DialogController=POWERSYS.PowerSysDialog  mask(Discrete PI Controller){Kp=2*pi*wcur*Lq, Ki=2*pi*wcur*R, Par_Limits=[V_max -V_max], Init=0, Ts=Ts}
      mask prompts: Kp "Proportional gain (Kp):"; Ki "Integral gain (Ki):"; Par_Limits "Output limits: [ Upper   Lower ]"; Init "Output initial value:"; Ts "Sample time:"
      mask help: This block implements a discrete PI controller.
      mask init:
      | UpperLimit=Par_Limits(1);
      | LowerLimit=Par_Limits(2);
      | power_initmask();
      mask Help: This block is part of a subset of blocks in the Extras library that does not have documentation associated with it, other than the block mask description.
      mask Display: disp('PI');
  Sum2 : Sum  Inputs=|+-
  Sum6 : Sum  Inputs=|++
  Out1 : Outport
  wires:
  In3/1 -> Sum2/2
  30iq/1(Out) -> Sum6/1  "ideal"
  Sum2/1 -> 30iq/1(Error)
  In1/1 -> Sum2/1
  Sum6/1 -> Out1/1

== system reduce_emf_load_fixed_v13/电流采样与矢量控制/Anti_Park ==
  thera : Inport
  Vq : Inport  Port=2
  Vd : Inport  Port=3
  Fcn : Fcn  Expr=cos(u[1])*u[2]-sin(u[1])*u[3]
  Fcn1 : Fcn  Expr=sin(u[1])*u[2]+cos(u[1])*u[3]
  Mux1 : Mux  Inputs=3
  Valpha : Outport
  Vbeta : Outport  Port=2
  wires:
  thera/1 -> Mux1/1
  Mux1/1 -> Fcn1/1, Fcn/1
  Vq/1 -> Mux1/3
  Fcn1/1 -> Vbeta/1
  Vd/1 -> Mux1/2
  Fcn/1 -> Valpha/1

== system reduce_emf_load_fixed_v13/电流采样与矢量控制/SVPWM ==
  Ualpha : Inport
  Ubeta : Inport  Port=2
  Rate Transition : RateTransition  Deterministic=off
  Rate Transition12 : RateTransition  Deterministic=off
  SVPWM : Subsystem
  P : Outport
  wires:
  Ualpha/1 -> Rate Transition/1
  Ubeta/1 -> Rate Transition12/1
  Rate Transition/1 -> SVPWM/1(alpha)
  Rate Transition12/1 -> SVPWM/2(beta)
  SVPWM/1(Pulse) -> P/1

== system reduce_emf_load_fixed_v13/反电动势观测与锁相环/锁相环1 ==
  Ed_hat : Inport
  Eq_hat : Inport  Port=2
  IF_sensorless_mode : Inport  Port=3
  MATLAB Function : MATLAB Function  TreatAsAtomicUnit=on
  theta : Outport
  we : Outport  Port=2
  id_offset : Outport  Port=3
  vfl_state : Outport  Port=4
  wires:
  Ed_hat/1 -> MATLAB Function/1(Ed_hat)
  Eq_hat/1 -> MATLAB Function/2(Eq_hat)
  MATLAB Function/1(theta) -> theta/1
  MATLAB Function/2(we) -> we/1
  IF_sensorless_mode/1 -> MATLAB Function/3(IF_sensorless_mode)
  MATLAB Function/3(id_offset) -> id_offset/1
  MATLAB Function/4(vfl_state) -> vfl_state/1
  [ID_sample_ack] -> MATLAB Function/4(sample_ack)

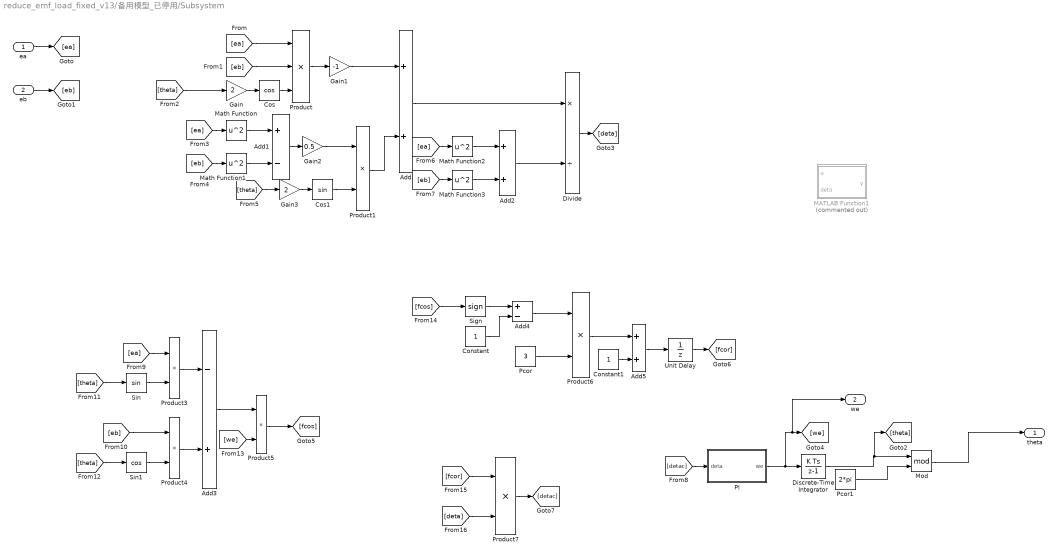
== system reduce_emf_load_fixed_v13/备用模型_已停用/Subsystem ==
  ea : Inport
  eb : Inport  Port=2
  Add : Sum
  Add1 : Sum  Inputs=+-
  Add2 : Sum
  Add3 : Sum  Inputs=-+
  Add4 : Sum  Inputs=+-
  Add5 : Sum
  Constant : Constant
  Constant1 : Constant
  Cos : Trigonometry  Operator=cos
  Cos1 : Trigonometry
  Discrete-Time Integrator : DiscreteIntegrator  SampleTime=-1  ICPrevOutput=DiscIntNeverNeededParam  ICPrevScaledInput=DiscIntNeverNeededParam
  Divide : Product  Inputs=*/
  Gain : Gain  Gain=2
  Gain1 : Gain  Gain=-1
  Gain2 : Gain  Gain=0.5
  Gain3 : Gain  Gain=2
  MATLAB Function1 : MATLAB Function  Commented=on  TreatAsAtomicUnit=on
  Math Function{,1..3} (4 alike) : Math  Operator=square
  Mod : Math  Operator=mod
  PI : Subsystem
  Pcor : Constant  Value=3
  Pcor1 : Constant  Value=2*pi
  Product : Product  Inputs=3
  Product{1,3..7} (6 alike) : Product
  Sign : Signum
  Sin : Trigonometry
  Sin1 : Trigonometry  Operator=cos
  Unit Delay : UnitDelay  SampleTime=-1  HasFrameUpgradeWarning=on
  theta : Outport
  we : Outport  Port=2
  wires:
  ea/1 -> [ea]
  eb/1 -> [eb]
  [ea] -> Product/1
  [eb] -> Product/2
  Cos/1 -> Product/3
  Gain/1 -> Cos/1
  [theta] -> Gain/1
  Product/1 -> Gain1/1
  Gain1/1 -> Add/1
  [ea] -> Math Function/1
  [eb] -> Math Function1/1
  Math Function/1 -> Add1/1
  Math Function1/1 -> Add1/2
  Add1/1 -> Gain2/1
  Gain2/1 -> Product1/1
  Product1/1 -> Add/2
  Cos1/1 -> Product1/2
  Gain3/1 -> Cos1/1
  [theta] -> Gain3/1
  Add/1 -> Divide/1
  Math Function3/1 -> Add2/2
  [ea] -> Math Function2/1
  [eb] -> Math Function3/1
  Math Function2/1 -> Add2/1
  [ea] -> Product3/1
  Sin/1 -> Product3/2
  [theta] -> Sin/1
  [eb] -> Product4/1
  [theta] -> Sin1/1
  Sin1/1 -> Product4/2
  Product3/1 -> Add3/1
  Product4/1 -> Add3/2
  Add3/1 -> Product5/1
  [we] -> Product5/2
  Product5/1 -> [fcos]
  [fcos] -> Sign/1
  Sign/1 -> Add4/1
  Constant/1 -> Add4/2
  Add4/1 -> Product6/1
  Pcor/1 -> Product6/2
  Product6/1 -> Add5/1
  Constant1/1 -> Add5/2
  Add5/1 -> Unit Delay/1
  [fcor] -> Product7/1
  [deta] -> Product7/2
  Product7/1 -> [detac]
  PI/1(we) -> Discrete-Time Integrator/1, we/1, [we]
  Discrete-Time Integrator/1 -> [theta], Mod/1
  Unit Delay/1 -> [fcor]
  Pcor1/1 -> Mod/2
  [detac] -> PI/1(deta)
  Add2/1 -> Divide/2
  Divide/1 -> [deta]
  Mod/1 -> theta/1

== system reduce_emf_load_fixed_v13/启动与速度控制/转速环/30speed ==
  note: Discrete PID Controller
  note: Pierre Giroux, Gilbert Sybille
      | Power System Simulation Laboratory
      | IREQ, Hydro-Quebc
  Error : Inport  SampleTime=Ts
  Add : Sum
  Add1 : Sum  Inputs=-+
  Discrete-Time Integrator : DiscreteIntegrator  InitialCondition=Init  SampleTime=Ts  UpperSaturationLimit=UpperLimit  LowerSaturationLimit=LowerLimit  ICPrevOutput=DiscIntNeverNeededParam  ICPrevScaledInput=DiscIntNeverNeededParam
  Kp1 : Gain  Gain=1/Kp  SaturateOnIntegerOverflow=on  SampleTime=Ts  OutDataTypeStr=Inherit: Same as input  ParamDataTypeStr=Inherit: Same as input
  Kp4 : Gain  Gain=Kp  SaturateOnIntegerOverflow=on  SampleTime=Ts  OutDataTypeStr=Inherit: Same as input  ParamDataTypeStr=Inherit: Same as input
  Kp5 : Gain  Gain=Ki  SaturateOnIntegerOverflow=on  SampleTime=Ts  OutDataTypeStr=Inherit: Same as input  ParamDataTypeStr=Inherit: Same as input
  Saturation2 : Saturate  UpperLimit=UpperLimit  LowerLimit=LowerLimit  SampleTime=Ts
  Sum6 : Sum  InputSameDT=on  SaturateOnIntegerOverflow=on  SampleTime=Ts  OutDataTypeStr=Inherit: Same as first input
  Zero-Order Hold : ZeroOrderHold  SampleTime=Ts
  Out : Outport  SampleTime=Ts  InitialOutput=0
  wires:
  Kp1/1 -> Add/2
  Add1/1 -> Kp1/1
  Add/1 -> Kp5/1
  Zero-Order Hold/1 -> Sum6/1
  Discrete-Time Integrator/1 -> Sum6/2
  Kp4/1 -> Zero-Order Hold/1
  Kp5/1 -> Discrete-Time Integrator/1
  Error/1 -> Kp4/1, Add/1
  Sum6/1 -> Saturation2/1, Add1/1
  Saturation2/1 -> Out/1, Add1/2

== system reduce_emf_load_fixed_v13/电流采样与矢量控制/d轴电流环/30id ==
  note: Discrete PID Controller
  note: Pierre Giroux, Gilbert Sybille
      | Power System Simulation Laboratory
      | IREQ, Hydro-Quebc
  Error : Inport  SampleTime=Ts
  Add : Sum
  Add1 : Sum  Inputs=-+
  Discrete-Time Integrator : DiscreteIntegrator  InitialCondition=Init  SampleTime=Ts  LimitOutput=on  UpperSaturationLimit=UpperLimit  LowerSaturationLimit=LowerLimit  ICPrevOutput=DiscIntNeverNeededParam  ICPrevScaledInput=DiscIntNeverNeededParam
  Kp1 : Gain  Gain=1/Kp  SaturateOnIntegerOverflow=on  SampleTime=Ts  OutDataTypeStr=Inherit: Same as input  ParamDataTypeStr=Inherit: Same as input
  Kp4 : Gain  Gain=Kp  SaturateOnIntegerOverflow=on  SampleTime=Ts  OutDataTypeStr=Inherit: Same as input  ParamDataTypeStr=Inherit: Same as input
  Kp5 : Gain  Gain=Ki  SaturateOnIntegerOverflow=on  SampleTime=Ts  OutDataTypeStr=Inherit: Same as input  ParamDataTypeStr=Inherit: Same as input
  Saturation2 : Saturate  UpperLimit=UpperLimit  LowerLimit=LowerLimit  SampleTime=Ts
  Scope : Scope  NumInputPorts=2
  Sum6 : Sum  InputSameDT=on  SaturateOnIntegerOverflow=on  SampleTime=Ts  OutDataTypeStr=Inherit: Same as first input
  Zero-Order Hold : ZeroOrderHold  SampleTime=Ts
  Out : Outport  SampleTime=Ts  InitialOutput=0
  wires:
  Error/1 -> Kp4/1, Add/1
  Kp5/1 -> Discrete-Time Integrator/1
  Discrete-Time Integrator/1 -> Scope/2, Sum6/2
  Kp4/1 -> Zero-Order Hold/1
  Kp1/1 -> Add/2
  Add1/1 -> Kp1/1
  Sum6/1 -> Add1/1, Saturation2/1
  Add/1 -> Kp5/1
  Saturation2/1 -> Add1/2, Out/1
  Zero-Order Hold/1 -> Scope/1, Sum6/1

== system reduce_emf_load_fixed_v13/电流采样与矢量控制/q轴电流环/30iq ==
  note: Discrete PID Controller
  note: Pierre Giroux, Gilbert Sybille
      | Power System Simulation Laboratory
      | IREQ, Hydro-Quebc
  Error : Inport  SampleTime=Ts
  Add : Sum
  Add1 : Sum  Inputs=-+
  Discrete-Time Integrator : DiscreteIntegrator  InitialCondition=Init  SampleTime=Ts  LimitOutput=on  UpperSaturationLimit=UpperLimit  LowerSaturationLimit=LowerLimit  ICPrevOutput=DiscIntNeverNeededParam  ICPrevScaledInput=DiscIntNeverNeededParam
  Kp1 : Gain  Gain=1/Kp  SaturateOnIntegerOverflow=on  SampleTime=Ts  OutDataTypeStr=Inherit: Same as input  ParamDataTypeStr=Inherit: Same as input
  Kp4 : Gain  Gain=Kp  SaturateOnIntegerOverflow=on  SampleTime=Ts  OutDataTypeStr=Inherit: Same as input  ParamDataTypeStr=Inherit: Same as input
  Kp5 : Gain  Gain=Ki  SaturateOnIntegerOverflow=on  SampleTime=Ts  OutDataTypeStr=Inherit: Same as input  ParamDataTypeStr=Inherit: Same as input
  Saturation2 : Saturate  UpperLimit=UpperLimit  LowerLimit=LowerLimit  SampleTime=Ts
  Scope : Scope  NumInputPorts=2
  Sum6 : Sum  InputSameDT=on  SaturateOnIntegerOverflow=on  SampleTime=Ts  OutDataTypeStr=Inherit: Same as first input
  Zero-Order Hold : ZeroOrderHold  SampleTime=Ts
  Out : Outport  SampleTime=Ts  InitialOutput=0
  wires:
  Zero-Order Hold/1 -> Scope/1, Sum6/1
  Discrete-Time Integrator/1 -> Scope/2, Sum6/2
  Kp4/1 -> Zero-Order Hold/1
  Kp5/1 -> Discrete-Time Integrator/1
  Sum6/1 -> Add1/1, Saturation2/1
  Error/1 -> Kp4/1, Add/1
  Saturation2/1 -> Add1/2, Out/1
  Add1/1 -> Kp1/1
  Add/1 -> Kp5/1
  Kp1/1 -> Add/2

== system reduce_emf_load_fixed_v13/电流采样与矢量控制/SVPWM/SVPWM ==
  alpha : Inport
  beta : Inport  Port=2
  Demux : Demux  Outputs=6
  N Caculate : Subsystem
  Repeating Sequence : simulink/Sources/Repeating Sequence  rep_seq_t=[0 0.5*Tpwm Tpwm]  rep_seq_y=[0 0.5*Tpwm 0]
  Sabc Pulse : Subsystem
  Scope : Scope  NumInputPorts=6
  Scope1 : Scope
  T1 T2 Caculate : Subsystem
  Tc Caculate : Subsystem
  Ts : Constant  Value=Tpwm
  "Udc " : Constant  Value=Vdc
  XYZ Caculate : Subsystem
  Pulse : Outport  VectorParamsAs1DForOutWhenUnconnected=off
  wires:
  beta/1 -> N Caculate/1(beta), XYZ Caculate/1(beta)
  alpha/1 -> N Caculate/2(alpha), XYZ Caculate/2(alpha)
  XYZ Caculate/1(X) -> T1 T2 Caculate/1(X)
  XYZ Caculate/2(Y) -> T1 T2 Caculate/2(Y)
  XYZ Caculate/3(Z) -> T1 T2 Caculate/3(Z)
  Ts/1 -> XYZ Caculate/3("Ts "), Tc Caculate/3(Ts), T1 T2 Caculate/5("Ts ")
  T1 T2 Caculate/1(T1) -> Tc Caculate/1(T1)
  T1 T2 Caculate/2(T2) -> Tc Caculate/2(T2)
  Tc Caculate/3(Tc3) -> Sabc Pulse/3(Tc3)
  Sabc Pulse/1("Pulse ") -> Demux/1, Pulse/1
  "Udc "/1 -> XYZ Caculate/4(Udc)
  Repeating Sequence/1 -> Sabc Pulse/4(Wave)
  Demux/1 -> Scope/1
  Demux/2 -> Scope/2
  Demux/3 -> Scope/3
  Demux/4 -> Scope/4
  Demux/5 -> Scope/5
  Demux/6 -> Scope/6
  N Caculate/1(N) -> Scope1/1, Tc Caculate/4(N), T1 T2 Caculate/4(N)
  Tc Caculate/2(Tc2) -> Sabc Pulse/2(Tc2)
  Tc Caculate/1(Tc1) -> Sabc Pulse/1(Tc1)

== system reduce_emf_load_fixed_v13/备用模型_已停用/Subsystem/PI ==
  deta : Inport
  Add : Sum
  Discrete-Time Integrator : DiscreteIntegrator  SampleTime=-1  ICPrevOutput=DiscIntNeverNeededParam  ICPrevScaledInput=DiscIntNeverNeededParam
  ki : Gain  Gain=wn^2
  kp : Gain  Gain=2*wn
  we : Outport
  wires:
  ki/1 -> Discrete-Time Integrator/1
  deta/1 -> kp/1, ki/1
  Discrete-Time Integrator/1 -> Add/1
  kp/1 -> Add/2
  Add/1 -> we/1

== system reduce_emf_load_fixed_v13/电流采样与矢量控制/SVPWM/SVPWM/N Caculate ==
  beta : Inport
  alpha : Inport  Port=2
  Add : Sum  Inputs=+-
  Add1 : Sum  Inputs=--
  Add2 : Sum  Inputs=+++
  Constant : Constant
  Constant1 : Constant  Value=0
  Gain : Gain  Gain=sqrt(3)/2
  Gain1 : Gain  Gain=1/2
  Gain2 : Gain  Gain=4
  Gain3 : Gain  Gain=2
  Gain4 : Gain
  MATLAB Function : MATLAB Function  TreatAsAtomicUnit=on
  Switch : Switch  Criteria=u2 > Threshold  SaturateOnIntegerOverflow=off  InputSameDT=off
  Switch1 : Switch  Criteria=u2 > Threshold  SaturateOnIntegerOverflow=off  InputSameDT=off
  Switch2 : Switch  Criteria=u2 > Threshold  SaturateOnIntegerOverflow=off  InputSameDT=off
  N : Outport  VectorParamsAs1DForOutWhenUnconnected=off
  wires:
  Switch/1 -> Gain4/1  "A"
  Add/1 -> Switch1/2
  Gain/1 -> Add1/1, Add/1
  Gain3/1 -> Add2/2
  Gain2/1 -> Add2/3
  Constant/1 -> Switch/1, Switch2/1, Switch1/1
  Add1/1 -> Switch2/2
  Gain1/1 -> Add1/2, Add/2
  Add2/1 -> MATLAB Function/1(u)
  Constant1/1 -> Switch2/3, Switch1/3, Switch/3
  Gain4/1 -> Add2/1
  beta/1 -> Switch/2, Gain1/1
  Switch2/1 -> Gain2/1  "C"
  Switch1/1 -> Gain3/1  "B"
  alpha/1 -> Gain/1
  MATLAB Function/1(y) -> N/1

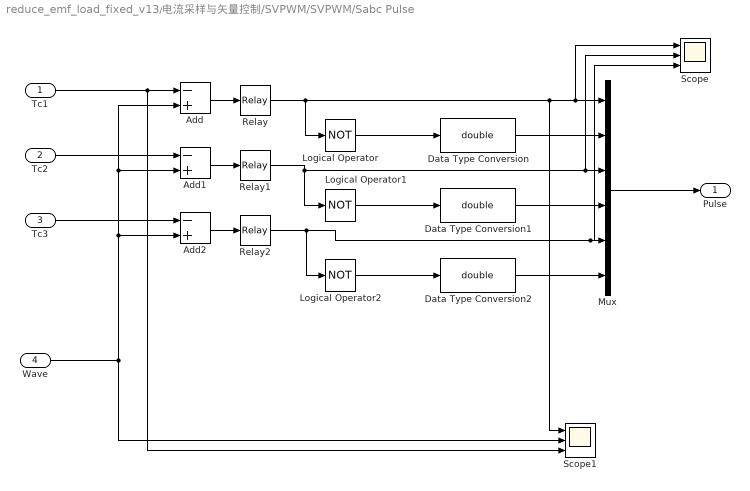
== system reduce_emf_load_fixed_v13/电流采样与矢量控制/SVPWM/SVPWM/Sabc Pulse ==
  Tc1 : Inport
  Tc2 : Inport  Port=2
  Tc3 : Inport  Port=3
  Wave : Inport  Port=4
  Add : Sum  Inputs=-+
  Add1 : Sum  Inputs=-+
  Add2 : Sum  Inputs=-+
  Data Type Conversion : DataTypeConversion  OutDataTypeStr=double  SaturateOnIntegerOverflow=off  RndMeth=Floor
  Data Type Conversion1 : DataTypeConversion  OutDataTypeStr=double  SaturateOnIntegerOverflow=off  RndMeth=Floor
  Data Type Conversion2 : DataTypeConversion  OutDataTypeStr=double  SaturateOnIntegerOverflow=off  RndMeth=Floor
  Logical Operator : Logic  Operator=NOT  AllPortsSameDT=off  OutDataTypeStr=boolean
  Logical Operator1 : Logic  Operator=NOT  AllPortsSameDT=off  OutDataTypeStr=boolean
  Logical Operator2 : Logic  Operator=NOT  AllPortsSameDT=off  OutDataTypeStr=boolean
  Mux : Mux  Inputs=6
  Relay : Relay
  Relay1 : Relay
  Relay2 : Relay
  Scope : Scope  NumInputPorts=3
  Scope1 : Scope  NumInputPorts=3
  "Pulse " : Outport  VectorParamsAs1DForOutWhenUnconnected=off
  wires:
  Add/1 -> Relay/1
  Add1/1 -> Relay1/1
  Wave/1 -> Add2/2, Add1/2, Add/2, Scope1/2
  Tc2/1 -> Add1/1
  Tc1/1 -> Scope1/3, Add/1
  Tc3/1 -> Add2/1
  Logical Operator/1 -> Data Type Conversion/1
  Logical Operator1/1 -> Data Type Conversion1/1
  Add2/1 -> Relay2/1
  Logical Operator2/1 -> Data Type Conversion2/1
  Mux/1 -> "Pulse "/1
  Relay/1 -> Scope1/1, Scope/1, Mux/1, Logical Operator/1
  Relay1/1 -> Scope/2, Mux/3, Logical Operator1/1
  Relay2/1 -> Logical Operator2/1, Scope/3, Mux/5
  Data Type Conversion/1 -> Mux/2
  Data Type Conversion1/1 -> Mux/4
  Data Type Conversion2/1 -> Mux/6

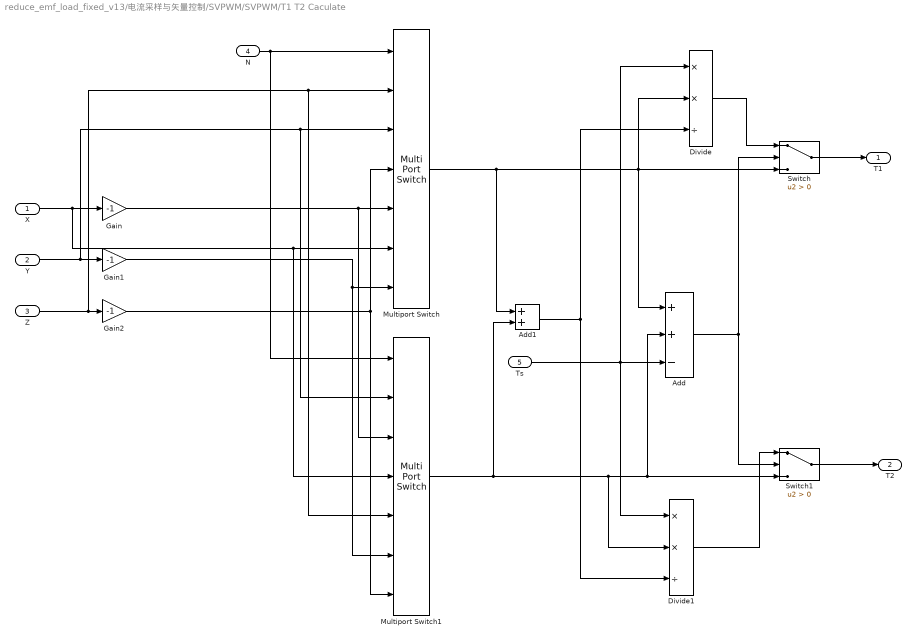
== system reduce_emf_load_fixed_v13/电流采样与矢量控制/SVPWM/SVPWM/T1 T2 Caculate ==
  X : Inport
  Y : Inport  Port=2
  Z : Inport  Port=3
  N : Inport  Port=4
  "Ts " : Inport  Port=5
  Add : Sum  Inputs=++-
  Add1 : Sum
  Divide : Product  Inputs=**/
  Divide1 : Product  Inputs=**/
  Gain : Gain  Gain=-1
  Gain1 : Gain  Gain=-1
  Gain2 : Gain  Gain=-1
  Multiport Switch : MultiPortSwitch  Inputs=6  SaturateOnIntegerOverflow=off  InputSameDT=off
  Multiport Switch1 : MultiPortSwitch  Inputs=6  SaturateOnIntegerOverflow=off  InputSameDT=off
  Switch : Switch  Criteria=u2 > Threshold  SaturateOnIntegerOverflow=off  InputSameDT=off
  Switch1 : Switch  Criteria=u2 > Threshold  SaturateOnIntegerOverflow=off  InputSameDT=off
  T1 : Outport  VectorParamsAs1DForOutWhenUnconnected=off
  T2 : Outport  Port=2  VectorParamsAs1DForOutWhenUnconnected=off
  wires:
  Y/1 -> Multiport Switch1/2, Multiport Switch/3, Gain1/1
  X/1 -> Multiport Switch1/4, Multiport Switch/6, Gain/1
  N/1 -> Multiport Switch/1, Multiport Switch1/1
  Z/1 -> Multiport Switch1/5, Multiport Switch/2, Gain2/1
  Gain2/1 -> Multiport Switch1/7, Multiport Switch/4
  Gain/1 -> Multiport Switch1/3, Multiport Switch/5
  Gain1/1 -> Multiport Switch1/6, Multiport Switch/7
  Multiport Switch/1 -> Add1/1, Divide/2, Add/1, Switch/3
  Multiport Switch1/1 -> Add1/2, Divide1/2, Add/2, Switch1/3
  "Ts "/1 -> Divide1/1, Divide/1, Add/3
  Add/1 -> Switch1/2, Switch/2
  Divide/1 -> Switch/1
  Add1/1 -> Divide/3, Divide1/3
  Switch/1 -> T1/1
  Switch1/1 -> T2/1
  Divide1/1 -> Switch1/1

== system reduce_emf_load_fixed_v13/电流采样与矢量控制/SVPWM/SVPWM/Tc Caculate ==
  T1 : Inport
  T2 : Inport  Port=2
  Ts : Inport  Port=3
  N : Inport  Port=4
  Multiport Switch : MultiPortSwitch  Inputs=6  SaturateOnIntegerOverflow=off  InputSameDT=off
  Multiport Switch1 : MultiPortSwitch  Inputs=6  SaturateOnIntegerOverflow=off  InputSameDT=off
  Multiport Switch2 : MultiPortSwitch  Inputs=6  SaturateOnIntegerOverflow=off  InputSameDT=off
  Mux : Mux  Inputs=3
  Scope : Scope  NumInputPorts=3
  Ta : Fcn  Expr=(u(3)-u(1)-u(2))/4
  Tb : Fcn  Expr=(u(3)-u(2)+u(1))/4
  Tc : Fcn  Expr=(u(3)+u(2)+u(1))/4
  Tc1 : Outport  VectorParamsAs1DForOutWhenUnconnected=off
  Tc2 : Outport  Port=2  VectorParamsAs1DForOutWhenUnconnected=off
  Tc3 : Outport  Port=3  VectorParamsAs1DForOutWhenUnconnected=off
  wires:
  T2/1 -> Mux/2
  T1/1 -> Mux/1
  Ts/1 -> Mux/3
  Mux/1 -> Tc/1, Ta/1, Tb/1
  N/1 -> Multiport Switch2/1, Multiport Switch1/1, Multiport Switch/1
  Ta/1 -> Multiport Switch2/7, Multiport Switch2/5, Multiport Switch/3, Multiport Switch/4, Multiport Switch1/6, Multiport Switch1/2
  Tb/1 -> Multiport Switch/7, Multiport Switch/2, Multiport Switch1/4, Multiport Switch2/6, Multiport Switch2/3, Multiport Switch1/5
  Tc/1 -> Multiport Switch2/4, Multiport Switch2/2, Multiport Switch1/7, Multiport Switch1/3, Multiport Switch/6, Multiport Switch/5
  Multiport Switch/1 -> Scope/1, Tc1/1
  Multiport Switch1/1 -> Scope/2, Tc2/1
  Multiport Switch2/1 -> Scope/3, Tc3/1

== system reduce_emf_load_fixed_v13/电流采样与矢量控制/SVPWM/SVPWM/XYZ Caculate ==
  beta : Inport
  alpha : Inport  Port=2
  "Ts " : Inport  Port=3
  Udc : Inport  Port=4
  Add : Sum
  Add1 : Sum  Inputs=-+
  Constant : Constant  Value=sqrt(3)
  Constant1 : Constant  Value=sqrt(3)/2
  Constant2 : Constant  Value=sqrt(3)/2
  Divide : Product  Inputs=***/
  Divide1 : Product  Inputs=***/
  Divide2 : Product  Inputs=***/
  Gain : Gain  Gain=sqrt(3)
  X : Outport  VectorParamsAs1DForOutWhenUnconnected=off
  Y : Outport  Port=2  VectorParamsAs1DForOutWhenUnconnected=off
  Z : Outport  Port=3  VectorParamsAs1DForOutWhenUnconnected=off
  wires:
  "Ts "/1 -> Divide2/1, Divide1/1, Divide/1
  Udc/1 -> Divide1/4, Divide2/4, Divide/4
  Constant/1 -> Divide/3
  beta/1 -> Add1/2, Add/2, Divide/2
  Constant2/1 -> Divide2/3
  Constant1/1 -> Divide1/3
  Add/1 -> Divide1/2
  Add1/1 -> Divide2/2
  Gain/1 -> Add1/1, Add/1
  alpha/1 -> Gain/1
  Divide1/1 -> Y/1
  Divide/1 -> X/1
  Divide2/1 -> Z/1
